simulink model "GuidanceLaw"  (R2023b)
settings: Solver=ode4  StartTime=0.0  StopTime=400  FixedStep=0.05  RelTol=1e-3
values from neighbouring files (symbols this model uses):
  APCMD_TYPE : value not decoded    [apDataDictionary.sldd]
  missionRoutePlan_struct = struct(      'validWpNum_u8', uint8(5),      'missionRoute_struct', repmat(wpDefault_struct, double(maxWpNum_u8), 1))    [initMissionRoutePlan_MC.m]
  MSSN_TYPE : value not decoded    [apDataDictionary.sldd]
  setPoint_struct = struct('lat_deg_d',double(31.200000),'lon_deg_d',double(121.500000),'alt_m_f',single(100),'yaw_deg_f',single(0))    [APTest.m]
undefined symbols (not defined in the file or in its folder): apParams
libraries: simulink x13, simulink_extras x3
(part 2 of 7)

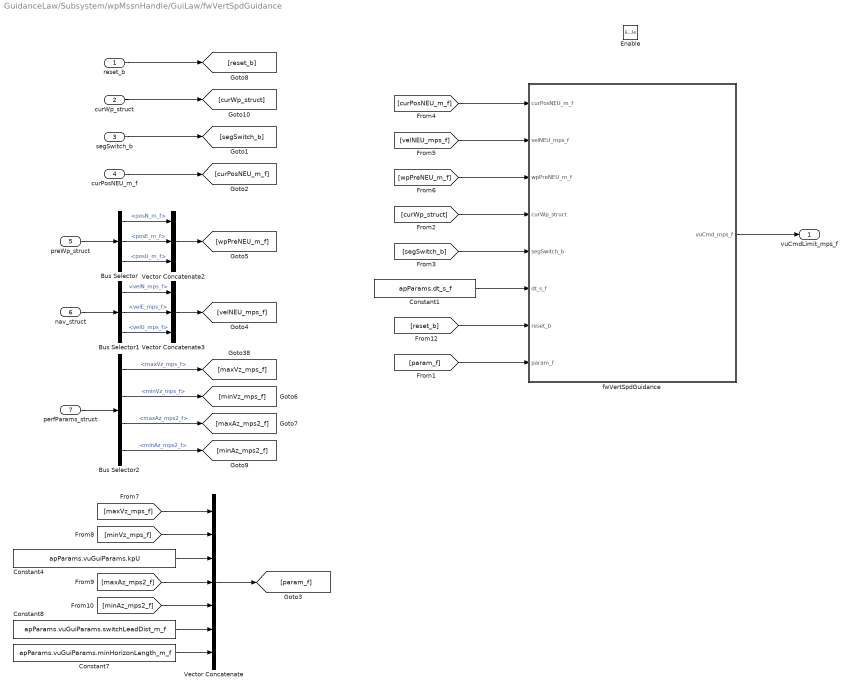
== system GuidanceLaw/Subsystem/wpMssnHandle/GuiLaw/fwVertSpdGuidance ==
  reset_b : Inport
  curWp_struct : Inport  Port=2
  segSwitch_b : Inport  Port=3
  curPosNEU_m_f : Inport  Port=4
  preWp_struct : Inport  Port=5
  nav_struct : Inport  Port=6
  perfParams_struct : Inport  Port=7
  Enable : EnablePort  StatesWhenEnabling=reset
  Bus Selector : BusSelector  OutputSignals=posN_m_f,posE_m_f,posU_m_f
  Bus Selector1 : BusSelector  OutputSignals=velN_mps_f,velE_mps_f,velU_mps_f
  Bus Selector2 : BusSelector  OutputSignals=maxVz_mps_f,minVz_mps_f,maxAz_mps2_f,minAz_mps2_f
  Constant1 : Constant  Value=apParams.dt_s_f  OutDataTypeStr=single
  Constant4 : Constant  Value=apParams.vuGuiParams.kpU  OutDataTypeStr=single
  Constant7 : Constant  Value=apParams.vuGuiParams.minHorizonLength_m_f  OutDataTypeStr=single
  Constant8 : Constant  Value=apParams.vuGuiParams.switchLeadDist_m_f  OutDataTypeStr=single
  Vector Concatenate : Concatenate  NumInputs=7
  Vector Concatenate2 : Concatenate  NumInputs=3
  Vector Concatenate3 : Concatenate  NumInputs=3
  fwVertSpdGuidance : MATLAB Function  TreatAsAtomicUnit=on
  vuCmdLimit_mps_f : Outport
  wires:
  fwVertSpdGuidance/1(vuCmd_mps_f) -> vuCmdLimit_mps_f/1
  Constant1/1 -> fwVertSpdGuidance/6(dt_s_f)
  reset_b/1 -> [reset_b]
  [reset_b] -> fwVertSpdGuidance/7(reset_b)
  Vector Concatenate/1 -> [param_f]
  [param_f] -> fwVertSpdGuidance/8(param_f)
  curWp_struct/1 -> [curWp_struct]
  [maxVz_mps_f] -> Vector Concatenate/1
  [minVz_mps_f] -> Vector Concatenate/2
  Constant4/1 -> Vector Concatenate/3
  [maxAz_mps2_f] -> Vector Concatenate/4
  [minAz_mps2_f] -> Vector Concatenate/5
  Constant7/1 -> Vector Concatenate/7
  Constant8/1 -> Vector Concatenate/6
  [curWp_struct] -> fwVertSpdGuidance/4(curWp_struct)
  segSwitch_b/1 -> [segSwitch_b]
  [segSwitch_b] -> fwVertSpdGuidance/5(segSwitch_b)
  curPosNEU_m_f/1 -> [curPosNEU_m_f]
  [curPosNEU_m_f] -> fwVertSpdGuidance/1(curPosNEU_m_f)
  [velNEU_mps_f] -> fwVertSpdGuidance/2(velNEU_mps_f)
  [wpPreNEU_m_f] -> fwVertSpdGuidance/3(wpPreNEU_m_f)
  preWp_struct/1 -> Bus Selector/1
  nav_struct/1 -> Bus Selector1/1
  Bus Selector/1 -> Vector Concatenate2/1  "<posN_m_f>"
  Bus Selector/2 -> Vector Concatenate2/2  "<posE_m_f>"
  Bus Selector/3 -> Vector Concatenate2/3  "<posU_m_f>"
  Vector Concatenate2/1 -> [wpPreNEU_m_f]
  Bus Selector1/1 -> Vector Concatenate3/1  "<velN_mps_f>"
  Bus Selector1/2 -> Vector Concatenate3/2  "<velE_mps_f>"
  Bus Selector1/3 -> Vector Concatenate3/3  "<velU_mps_f>"
  Vector Concatenate3/1 -> [velNEU_mps_f]
  perfParams_struct/1 -> Bus Selector2/1
  Bus Selector2/1 -> [maxVz_mps_f]  "<maxVz_mps_f>"
  Bus Selector2/2 -> [minVz_mps_f]  "<minVz_mps_f>"
  Bus Selector2/3 -> [maxAz_mps2_f]  "<maxAz_mps2_f>"
  Bus Selector2/4 -> [minAz_mps2_f]  "<minAz_mps2_f>"

== system GuidanceLaw/Subsystem/wpMssnHandle/GuiLaw/guiLawSelect ==
  flightPhase_enum : Inport
  preWp_struct : Inport  Port=2
  curWp_struct : Inport  Port=3
  guiLawSelect : MATLAB Function  TreatAsAtomicUnit=on
  guiLawType_u8 : Outport
  fwL1LineGui_b : Outport  Port=2
  fwL1CirGui_b : Outport  Port=3
  fwAirSpdGui_b : Outport  Port=4
  fwVertSpdGui_b : Outport  Port=5
  mcSpdGui_b : Outport  Port=6
  yawGui_b : Outport  Port=7
  segMssnType_u8 : Outport  Port=8
  tiltEnable_b : Outport  Port=9
  wires:
  guiLawSelect/1(guiLawType_u8) -> [guiLawType_u8]
  guiLawSelect/2(fwL1LineGui_b) -> [fwL1LineGui_b]
  guiLawSelect/3(fwL1CirGui_b) -> [fwL1CirGui_b]
  guiLawSelect/4(fwAirSpdGui_b) -> [fwAirSpdGui_b]
  guiLawSelect/5(fwVertSpdGui_b) -> [fwVertSpdGui_b]
  guiLawSelect/6(mcSpdGui_b) -> [mcSpdGui_b]
  guiLawSelect/7(yawGui_b) -> [yawGui_b]
  [flightPhase_enum] -> guiLawSelect/1(flightPhase_enum)
  [preWp_struct] -> guiLawSelect/2(preWp_struct)
  [curWp_struct] -> guiLawSelect/3(curWp_struct)
  flightPhase_enum/1 -> [flightPhase_enum]
  preWp_struct/1 -> [preWp_struct]
  curWp_struct/1 -> [curWp_struct]
  [guiLawType_u8] -> guiLawType_u8/1
  [fwL1LineGui_b] -> fwL1LineGui_b/1
  [fwL1CirGui_b] -> fwL1CirGui_b/1
  [fwAirSpdGui_b] -> fwAirSpdGui_b/1
  [fwVertSpdGui_b] -> fwVertSpdGui_b/1
  [mcSpdGui_b] -> mcSpdGui_b/1
  [yawGui_b] -> yawGui_b/1
  guiLawSelect/8(segMssnType_u8) -> [segMssnType_u8]
  [segMssnType_u8] -> segMssnType_u8/1
  guiLawSelect/9(tiltEnable_b) -> [tiltEnable_b]
  [tiltEnable_b] -> tiltEnable_b/1

== system GuidanceLaw/Subsystem/wpMssnHandle/GuiLaw/invaildGuidance ==
  nav_struct : Inport
  Bus Selector : BusSelector  OutputSignals=velN_mps_f,velE_mps_f,velU_mps_f,roll_deg_f,pitch_deg_f,yaw_deg_f
  NE2Body : Subsystem
  vuCmd_mps_f : Outport
  rollCmd_deg_f : Outport  Port=2
  pitchCmd_deg_f : Outport  Port=3
  yawCmd_deg_f : Outport  Port=4
  vyCmd_mps_f : Outport  Port=5
  vxCmd_mps_f : Outport  Port=6
  wires:
  nav_struct/1 -> Bus Selector/1
  Bus Selector/3 -> vuCmd_mps_f/1  "<velU_mps_f>"
  Bus Selector/4 -> rollCmd_deg_f/1  "<roll_deg_f>"
  Bus Selector/5 -> pitchCmd_deg_f/1  "<pitch_deg_f>"
  Bus Selector/6 -> [curYaw_deg_f], yawCmd_deg_f/1  "<yaw_deg_f>"
  Bus Selector/1 -> [curVn_mps_f]  "<velN_mps_f>"
  Bus Selector/2 -> [curVe_mps_f]  "<velE_mps_f>"
  NE2Body/1(vxCmd_mps_f) -> vxCmd_mps_f/1  "vxCmd_mps_f"
  NE2Body/2(vyCmd_mps_f) -> vyCmd_mps_f/1  "vyCmd_mps_f"
  [curYaw_deg_f] -> NE2Body/1(curYaw_deg_f)
  [curVe_mps_f] -> NE2Body/3(curVe_mps_f)
  [curVn_mps_f] -> NE2Body/2(curVn_mps_f)

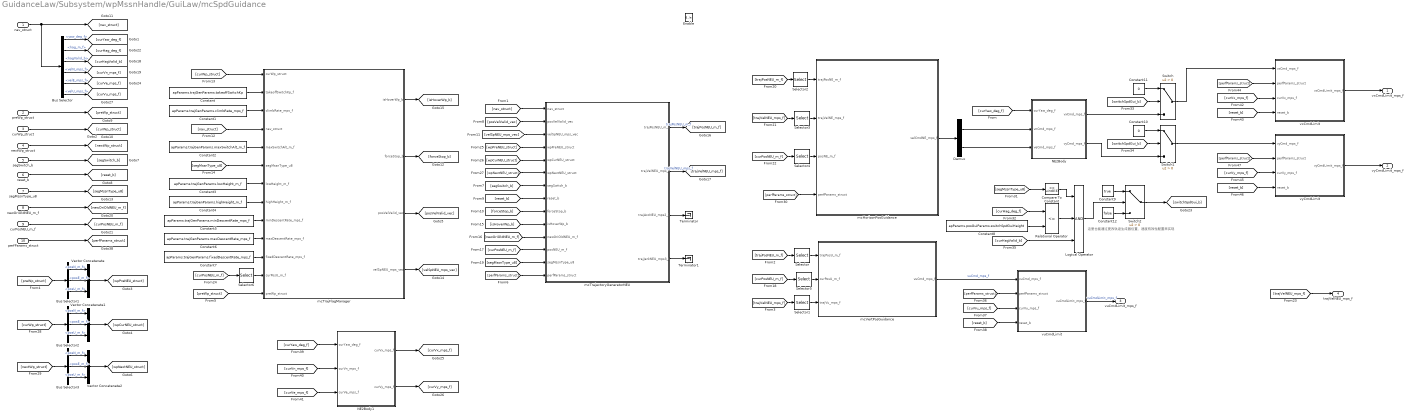
== system GuidanceLaw/Subsystem/wpMssnHandle/GuiLaw/mcSpdGuidance ==
  note: 这里也能通过更改轨迹生成器位置、速度有效性配置来实现
  nav_struct : Inport
  preWp_struct : Inport  Port=2
  curWp_struct : Inport  Port=3
  nextWp_struct : Inport  Port=4
  segSwitch_b : Inport  Port=5
  reset_b : Inport  Port=6
  segMssnType_u8 : Inport  Port=7
  newOriOldNEU_m_f : Inport  Port=8
  curPosNEU_m_f : Inport  Port=9
  perfParams_struct : Inport  Port=10
  Enable : EnablePort  StatesWhenEnabling=reset
  Bus Selector : BusSelector  OutputSignals=yaw_deg_f,hag_m_f,hagValid_b,velN_mps_f,velE_mps_f,velU_mps_f
  Bus Selector1 : BusSelector  OutputSignals=posN_m_f,posE_m_f,posU_m_f
  Bus Selector2 : BusSelector  OutputSignals=posN_m_f,posE_m_f,posU_m_f
  Bus Selector3 : BusSelector  OutputSignals=posN_m_f,posE_m_f,posU_m_f
  Compare To Constant : simulink/Logic and Bit Operations/Compare To Constant  relop===  const=uint8(3)  OutDataTypeStr=boolean
  Constant : Constant  Value=apParams.trajGenParams.takeoffSwitchKp  OutDataTypeStr=single
  Constant1 : Constant  Value=apParams.trajGenParams.climbRate_mps_f  OutDataTypeStr=single
  Constant10 : Constant  Value=0  OutDataTypeStr=single
  Constant11 : Constant  Value=0  OutDataTypeStr=single
  Constant12 : Constant  Value=false  OutDataTypeStr=boolean
  Constant2 : Constant  Value=apParams.trajGenParams.maxSwitchAlt_m_f  OutDataTypeStr=single
  Constant3 : Constant  Value=apParams.trajGenParams.lowHeight_m_f  OutDataTypeStr=single
  Constant4 : Constant  Value=apParams.trajGenParams.highHeight_m_f  OutDataTypeStr=single
  Constant5 : Constant  Value=apParams.trajGenParams.minDescentRate_mps_f  OutDataTypeStr=single
  Constant6 : Constant  Value=apParams.trajGenParams.maxDescentRate_mps_f  OutDataTypeStr=single
  Constant7 : Constant  Value=apParams.trajGenParams.fixedDescentRate_mps_f  OutDataTypeStr=single
  Constant8 : Constant  Value=apParams.posGuiParams.switchSpdGuiHeight  OutDataTypeStr=single
  Constant9 : Constant  Value=true  OutDataTypeStr=boolean
  Demux : Demux  Outputs=2
  Logical Operator : Logic  Inputs=3  AllPortsSameDT=off  OutDataTypeStr=boolean
  NE2Body : Subsystem
  NE2Body1 : Subsystem
  Relational Operator : RelationalOperator  Operator=<=  OutDataTypeStr=boolean  RndMeth=Simplest  InputSameDT=off
  Selector{,1,5..6} (4 alike) : Selector  InputPortWidth=3  IndexOptions=Index vector (dialog)  Indices=3  OutputSizes=1
  Selector2 : Selector  InputPortWidth=3  IndexOptions=Index vector (dialog)  Indices=[1 2]  OutputSizes=1
  Selector3 : Selector  InputPortWidth=3  IndexOptions=Index vector (dialog)  Indices=[1 2]  OutputSizes=1
  Selector4 : Selector  InputPortWidth=3  IndexOptions=Index vector (dialog)  Indices=[1 2]  OutputSizes=1
  Switch : Switch  Criteria=u2 > Threshold  SaturateOnIntegerOverflow=off  InputSameDT=off
  Switch1 : Switch  Criteria=u2 > Threshold  SaturateOnIntegerOverflow=off  InputSameDT=off
  Switch2 : Switch  Criteria=u2 > Threshold  SaturateOnIntegerOverflow=off  InputSameDT=off
  Terminator : Terminator
  Terminator1 : Terminator
  Vector Concatenate : Concatenate  NumInputs=3
  Vector Concatenate1 : Concatenate  NumInputs=3
  Vector Concatenate2 : Concatenate  NumInputs=3
  mcHorizonPosGuidance : Subsystem
  mcTrajFlagManager : MATLAB Function  TreatAsAtomicUnit=on
  mcTrajectoryGeneratorNEU : Subsystem
  mcVertPosGuidance : Subsystem
  vuCmdLimit : Subsystem
  vxCmdLimit : Subsystem
  vyCmdLimit : Subsystem
  vxCmdLimit_mps_f : Outport
  vyCmdLimit_mps_f : Outport  Port=2
  vuCmdLimit_mps_f : Outport  Port=3
  trajVelNEU_mps_f : Outport  Port=4
  wires:
  mcVertPosGuidance/1(vuCmd_mps_f) -> vuCmdLimit/1(vuCmd_mps_f)  "vuCmd_mps_f"
  NE2Body/1(vxCmd_mps_f) -> Switch/3
  mcHorizonPosGuidance/1(velCmdNE_mps_f) -> Demux/1
  Demux/1 -> NE2Body/2(vnCmd_mps_f)
  Demux/2 -> NE2Body/3(veCmd_mps_f)
  nav_struct/1 -> Bus Selector/1, [nav_struct]
  Bus Selector/1 -> [curYaw_deg_f]  "<yaw_deg_f>"
  [curYaw_deg_f] -> NE2Body/1(curYaw_deg_f)
  curWp_struct/1 -> [curWp_struct]
  preWp_struct/1 -> [preWp_struct]
  nextWp_struct/1 -> [nextWp_struct]
  [nav_struct] -> mcTrajectoryGeneratorNEU/1(nav_struct)
  segSwitch_b/1 -> [segSwitch_b]
  [segSwitch_b] -> mcTrajectoryGeneratorNEU/7(segSwitch_b)
  reset_b/1 -> [reset_b]
  [reset_b] -> mcTrajectoryGeneratorNEU/8(reset_b)
  [posVelValid_vec] -> mcTrajectoryGeneratorNEU/2(posVelValid_vec)
  mcTrajFlagManager/3(posVelValid_vec) -> [posVelValid_vec]
  [forceStop_b] -> mcTrajectoryGeneratorNEU/9(forceStop_b)
  [velSpNEU_mps_vec] -> mcTrajectoryGeneratorNEU/3(velSpNEU_mps_vec)
  [nav_struct] -> mcTrajFlagManager/4(nav_struct)
  [curWp_struct] -> mcTrajFlagManager/1(curWp_struct)
  Constant/1 -> mcTrajFlagManager/2(takeoffSwitchKp_f)
  Constant1/1 -> mcTrajFlagManager/3(climbRate_mps_f)
  Constant2/1 -> mcTrajFlagManager/5(maxSwitchAlt_m_f)
  mcTrajFlagManager/2(forceStop_b) -> [forceStop_b]
  segMssnType_u8/1 -> [segMssnType_u8]
  [segMssnType_u8] -> mcTrajFlagManager/6(segMssnType_u8)
  mcTrajFlagManager/4(velSpNEU_mps_vec) -> [velSpNEU_mps_vec]
  Constant3/1 -> mcTrajFlagManager/7(lowHeight_m_f)
  Constant4/1 -> mcTrajFlagManager/8(highHeight_m_f)
  Constant5/1 -> mcTrajFlagManager/9(minDescentRate_mps_f)
  Constant6/1 -> mcTrajFlagManager/10(maxDescentRate_mps_f)
  Constant7/1 -> mcTrajFlagManager/11(fixedDescentRate_mps_f)
  mcTrajFlagManager/1(isHoverWp_b) -> [isHoverWp_b]
  [isHoverWp_b] -> mcTrajectoryGeneratorNEU/10(isHoverWp_b)
  [newOriOldNEU_m_f] -> mcTrajectoryGeneratorNEU/11(newOriOldNEU_m_f)
  [curPosNEU_m_f] -> mcTrajectoryGeneratorNEU/12(posNEU_m_f)
  mcTrajectoryGeneratorNEU/1(trajPosNEU_m_f) -> [trajPosNEU_m_f]  "trajPosNEU_m_f"
  mcTrajectoryGeneratorNEU/2(trajVelNEU_mps_f) -> [trajVelNEU_mps_f]  "trajVelNEU_mps_f"
  mcTrajectoryGeneratorNEU/3(trajAccNEU_mps2_f) -> Terminator/1
  mcTrajectoryGeneratorNEU/4(trajJerkNEU_mps3_f) -> Terminator1/1
  newOriOldNEU_m_f/1 -> [newOriOldNEU_m_f]
  curPosNEU_m_f/1 -> [curPosNEU_m_f]
  [trajPosNEU_m_f] -> Selector/1
  Selector/1 -> mcVertPosGuidance/1(trajPosU_m_f)
  [trajVelNEU_mps_f] -> Selector1/1
  Selector1/1 -> mcVertPosGuidance/3(trajVu_mps_f)
  [curPosNEU_m_f] -> Selector5/1
  [segMssnType_u8] -> mcTrajectoryGeneratorNEU/13(segMssnType_u8)
  [trajPosNEU_m_f] -> Selector2/1
  Selector2/1 -> mcHorizonPosGuidance/1(trajPosNE_m_f)
  [trajVelNEU_mps_f] -> Selector3/1
  Selector3/1 -> mcHorizonPosGuidance/2(trajVelNE_mps_f)
  [curPosNEU_m_f] -> Selector4/1
  Selector4/1 -> mcHorizonPosGuidance/3(posNE_m_f)
  [trajVelNEU_mps_f] -> trajVelNEU_mps_f/1
  Selector5/1 -> mcVertPosGuidance/2(curPosU_m_f)
  [curPosNEU_m_f] -> Selector6/1
  Selector6/1 -> mcTrajFlagManager/12(curPosU_m_f)
  [preWp_struct] -> Bus Selector1/1
  Bus Selector1/1 -> Vector Concatenate/1  "<posN_m_f>"
  Bus Selector1/2 -> Vector Concatenate/2  "<posE_m_f>"
  Bus Selector1/3 -> Vector Concatenate/3  "<posU_m_f>"
  Vector Concatenate/1 -> [wpPreNEU_struct]
  [wpPreNEU_struct] -> mcTrajectoryGeneratorNEU/4(wpPreNEU_struct)
  [wpCurNEU_struct] -> mcTrajectoryGeneratorNEU/5(wpCurNEU_struct)
  [wpNextNEU_struct] -> mcTrajectoryGeneratorNEU/6(wpNextNEU_struct)
  Bus Selector2/3 -> Vector Concatenate1/3  "<posU_m_f>"
  Bus Selector2/2 -> Vector Concatenate1/2  "<posE_m_f>"
  Bus Selector2/1 -> Vector Concatenate1/1  "<posN_m_f>"
  Vector Concatenate1/1 -> [wpCurNEU_struct]
  [curWp_struct] -> Bus Selector2/1
  Bus Selector3/2 -> Vector Concatenate2/2  "<posE_m_f>"
  [nextWp_struct] -> Bus Selector3/1
  Bus Selector3/1 -> Vector Concatenate2/1  "<posN_m_f>"
  Bus Selector3/3 -> Vector Concatenate2/3  "<posU_m_f>"
  Vector Concatenate2/1 -> [wpNextNEU_struct]
  [preWp_struct] -> mcTrajFlagManager/13(preWp_struct)
  perfParams_struct/1 -> [perfParams_struct]
  [perfParams_struct] -> mcTrajectoryGeneratorNEU/14(perfParams_struct)
  [perfParams_struct] -> mcHorizonPosGuidance/4(perfParams_struct)
  Switch/1 -> vxCmdLimit/1(vxCmd_mps_f)
  NE2Body/2(vyCmd_mps_f) -> Switch1/3
  Constant10/1 -> Switch1/1
  Constant11/1 -> Switch/1
  [segMssnType_u8] -> Compare To Constant/1
  Compare To Constant/1 -> Logical Operator/1
  [curHag_deg_f] -> Relational Operator/1
  Bus Selector/2 -> [curHag_deg_f]  "<hag_m_f>"
  Constant8/1 -> Relational Operator/2
  Relational Operator/1 -> Logical Operator/2
  Logical Operator/1 -> Switch2/2
  Constant9/1 -> Switch2/1
  Constant12/1 -> Switch2/3
  Switch2/1 -> [switchSpdGui_b]
  [switchSpdGui_b] -> Switch/2
  [switchSpdGui_b] -> Switch1/2
  Bus Selector/3 -> [curHagValid_b]  "<hagValid_b>"
  [curHagValid_b] -> Logical Operator/3
  vuCmdLimit/1(vuCmdLimit_mps_f) -> vuCmdLimit_mps_f/1  "vuCmdLimit_mps_f"
  [perfParams_struct] -> vuCmdLimit/2(perfParams_struct)
  [curVu_mps_f] -> vuCmdLimit/3(curVu_mps_f)
  [reset_b] -> vuCmdLimit/4(reset_b)
  vxCmdLimit/1(vxCmdLimit_mps_f) -> vxCmdLimit_mps_f/1
  [curYaw_deg_f] -> NE2Body1/1(curYaw_deg_f)
  Bus Selector/4 -> [curVn_mps_f]  "<velN_mps_f>"
  Bus Selector/5 -> [curVe_mps_f]  "<velE_mps_f>"
  [curVn_mps_f] -> NE2Body1/2(curVn_mps_f)
  [curVe_mps_f] -> NE2Body1/3(curVe_mps_f)
  NE2Body1/1(curVx_mps_f) -> [curVx_mps_f]
  NE2Body1/2(curVy_mps_f) -> [curVy_mps_f]
  [curVx_mps_f] -> vxCmdLimit/3(curVx_mps_f)
  [reset_b] -> vxCmdLimit/4(reset_b)
  [perfParams_struct] -> vxCmdLimit/2(perfParams_struct)
  [reset_b] -> vyCmdLimit/4(reset_b)
  [curVy_mps_f] -> vyCmdLimit/3(curVy_mps_f)
  [perfParams_struct] -> vyCmdLimit/2(perfParams_struct)
  Switch1/1 -> vyCmdLimit/1(vyCmd_mps_f)
  vyCmdLimit/1(vyCmdLimit_mps_f) -> vyCmdLimit_mps_f/1
  Bus Selector/6 -> [curVu_mps_f]  "<velU_mps_f>"

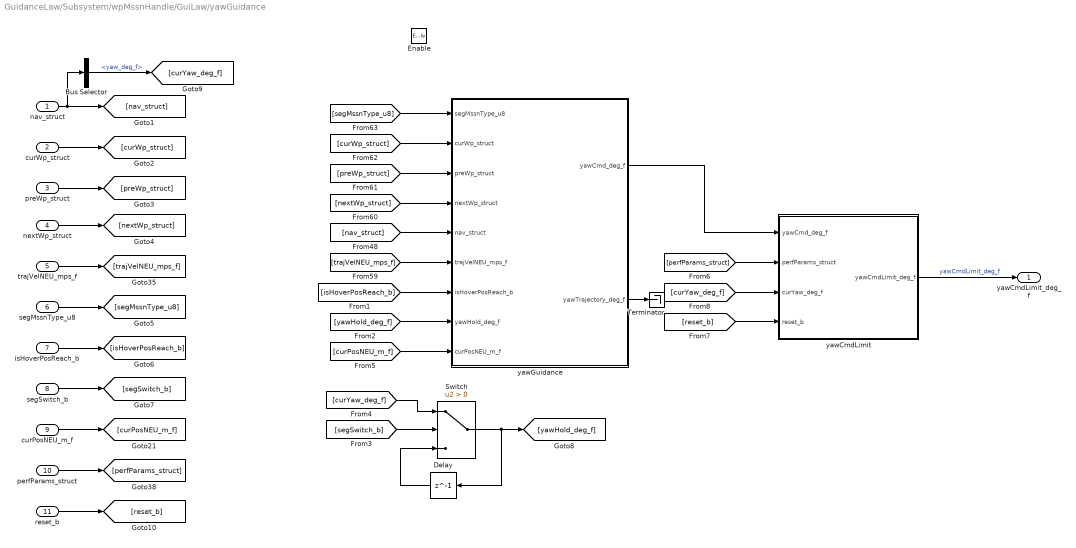
== system GuidanceLaw/Subsystem/wpMssnHandle/GuiLaw/yawGuidance ==
  nav_struct : Inport
  curWp_struct : Inport  Port=2
  preWp_struct : Inport  Port=3
  nextWp_struct : Inport  Port=4
  trajVelNEU_mps_f : Inport  Port=5
  segMssnType_u8 : Inport  Port=6
  isHoverPosReach_b : Inport  Port=7
  segSwitch_b : Inport  Port=8
  curPosNEU_m_f : Inport  Port=9
  perfParams_struct : Inport  Port=10
  reset_b : Inport  Port=11
  Enable : EnablePort  StatesWhenEnabling=reset
  Bus Selector : BusSelector  OutputSignals=yaw_deg_f
  Delay : Delay  DelayLength=1
  Switch : Switch  Criteria=u2 > Threshold  SaturateOnIntegerOverflow=off  InputSameDT=off
  Terminator : Terminator
  yawCmdLimit : Subsystem
  yawGuidance : MATLAB Function  TreatAsAtomicUnit=on
  yawCmdLimit_deg_f : Outport
  wires:
  trajVelNEU_mps_f/1 -> [trajVelNEU_mps_f]
  nav_struct/1 -> Bus Selector/1, [nav_struct]
  curWp_struct/1 -> [curWp_struct]
  preWp_struct/1 -> [preWp_struct]
  nextWp_struct/1 -> [nextWp_struct]
  segMssnType_u8/1 -> [segMssnType_u8]
  [nav_struct] -> yawGuidance/5(nav_struct)
  [nextWp_struct] -> yawGuidance/4(nextWp_struct)
  [preWp_struct] -> yawGuidance/3(preWp_struct)
  [curWp_struct] -> yawGuidance/2(curWp_struct)
  [segMssnType_u8] -> yawGuidance/1(segMssnType_u8)
  [trajVelNEU_mps_f] -> yawGuidance/6(trajVelNEU_mps_f)
  isHoverPosReach_b/1 -> [isHoverPosReach_b]
  [isHoverPosReach_b] -> yawGuidance/7(isHoverPosReach_b)
  segSwitch_b/1 -> [segSwitch_b]
  [yawHold_deg_f] -> yawGuidance/8(yawHold_deg_f)
  [segSwitch_b] -> Switch/2
  Switch/1 -> Delay/1, [yawHold_deg_f]
  Bus Selector/1 -> [curYaw_deg_f]  "<yaw_deg_f>"
  [curYaw_deg_f] -> Switch/1
  Delay/1 -> Switch/3
  curPosNEU_m_f/1 -> [curPosNEU_m_f]
  [curPosNEU_m_f] -> yawGuidance/9(curPosNEU_m_f)
  yawCmdLimit/1(yawCmdLimit_deg_f) -> yawCmdLimit_deg_f/1  "yawCmdLimit_deg_f"
  yawGuidance/1(yawCmd_deg_f) -> yawCmdLimit/1(yawCmd_deg_f)
  perfParams_struct/1 -> [perfParams_struct]
  [perfParams_struct] -> yawCmdLimit/2(perfParams_struct)
  reset_b/1 -> [reset_b]
  [reset_b] -> yawCmdLimit/4(reset_b)
  [curYaw_deg_f] -> yawCmdLimit/3(curYaw_deg_f)
  yawGuidance/2(yawTrajectory_deg_f) -> Terminator/1

== system GuidanceLaw/Subsystem/wpMssnHandle/WaypointArrivalState/cirJudge ==
  curPosNEU_m_f : Inport
  curWp_struct : Inport  Port=2
  nextWp_struct : Inport  Port=3
  reset_b : Inport  Port=4
  Enable : EnablePort  StatesWhenEnabling=reset
  Bus Selector1 : BusSelector  OutputSignals=posN_m_f,posE_m_f,posU_m_f,timeOrCount_u16,arrivalCond_u8
  Bus Selector2 : BusSelector  OutputSignals=posN_m_f,posE_m_f,posU_m_f
  Constant1 : Constant  Value=apParams.cirJudge.cirAltTolerance_m_f  OutDataTypeStr=single
  Constant21 : Constant  Value=apParams.dt_s_f  OutDataTypeStr=single
  Constant5 : Constant  Value=apParams.cirJudge.cirExitTolerance_deg_f  OutDataTypeStr=single
  MATLAB Function : MATLAB Function  TreatAsAtomicUnit=on
  MATLAB Function1 : MATLAB Function  Commented=on  TreatAsAtomicUnit=on
  Vector Concatenate1 : Concatenate  NumInputs=3
  Vector Concatenate2 : Concatenate  NumInputs=3
  cirJudge_b : Outport
  wires:
  MATLAB Function/1(cirJudge_b) -> cirJudge_b/1
  curPosNEU_m_f/1 -> MATLAB Function/1(curPosNEU_m_f)
  nextWp_struct/1 -> Bus Selector2/1
  Bus Selector1/1 -> Vector Concatenate1/1  "<posN_m_f>"
  Bus Selector1/2 -> Vector Concatenate1/2  "<posE_m_f>"
  Vector Concatenate1/1 -> [curWpNEU_m_f]
  Bus Selector2/2 -> Vector Concatenate2/2  "<posE_m_f>"
  Vector Concatenate2/1 -> [nextWpNEU_m_f]
  Bus Selector2/1 -> Vector Concatenate2/1  "<posN_m_f>"
  curWp_struct/1 -> Bus Selector1/1
  [curWpNEU_m_f] -> MATLAB Function/2(curWpNEU_m_f)
  [nextWpNEU_m_f] -> MATLAB Function/3(nextWpNEU_m_f)
  reset_b/1 -> MATLAB Function/9(reset_b)
  Constant5/1 -> MATLAB Function/6(cirExitTolerance_deg_f)
  Constant21/1 -> MATLAB Function/8(dt_s_f)
  Constant1/1 -> MATLAB Function/7(cirAltTolerance_m_f)
  Bus Selector1/4 -> [timeOrCount_u16]  "<timeOrCount_u16>"
  Bus Selector1/5 -> [arrivalCond_u8]  "<arrivalCond_u8>"
  [arrivalCond_u8] -> MATLAB Function/4(arrivalCond_u8)
  [timeOrCount_u16] -> MATLAB Function/5(timeOrCount_u16)
  Bus Selector1/3 -> Vector Concatenate1/3  "<posU_m_f>"
  Bus Selector2/3 -> Vector Concatenate2/3  "<posU_m_f>"

== system GuidanceLaw/Subsystem/wpMssnHandle/WaypointArrivalState/fwLineJudge ==
  curPosNEU_m_f : Inport
  reset_b : Inport  Port=2
  preWp_struct : Inport  Port=3
  curWp_struct : Inport  Port=4
  nextWp_struct : Inport  Port=5
  Enable : EnablePort  StatesWhenEnabling=reset
  Constant1 : Constant  Value=apParams.fwLineJudge.minJudgeDist_m_f  OutDataTypeStr=single
  Constant2 : Constant  Value=apParams.fwLineJudge.maxJudgeDist_m_f  OutDataTypeStr=single
  Constant3 : Constant  Value=apParams.fwLineJudge.segmentLimitRatio_f  OutDataTypeStr=single
  Constant4 : Constant  Value=apParams.G_mps2_f  OutDataTypeStr=single
  Constant5 : Constant  Value=apParams.fwLineJudge.effectRollRate_dps_f  OutDataTypeStr=single
  Constant6 : Constant  Value=apParams.airSpdGuiParams.cruiseAirSpd_mps_f  OutDataTypeStr=single
  Constant7 : Constant  Value=apParams.fwLineJudge.turnRollPlan_deg_f  OutDataTypeStr=single
  Constant8 : Constant  Value=apParams.fwLineJudge.judgeDistMargin_f  OutDataTypeStr=single
  JudgeAlgorithm : MATLAB Function  TreatAsAtomicUnit=on
  Selector : Selector  InputPortWidth=3  IndexOptions=Index vector (dialog)  Indices=[1 2]  OutputSizes=1
  fwLineJudge_b : Outport
  wires:
  JudgeAlgorithm/1(fwLineJudge_b) -> fwLineJudge_b/1
  reset_b/1 -> JudgeAlgorithm/11(reset_b)
  Constant3/1 -> JudgeAlgorithm/10(segmentLimitRatio_f)
  Constant2/1 -> JudgeAlgorithm/9(maxJudgeDist_m_f)
  Constant1/1 -> JudgeAlgorithm/8(minJudgeDist_m_f)
  Constant5/1 -> JudgeAlgorithm/6(effectRollRate_dps_f)
  Constant4/1 -> JudgeAlgorithm/12(G_mps2_f)
  Selector/1 -> JudgeAlgorithm/1(curPosNE_m_f)
  curPosNEU_m_f/1 -> Selector/1
  preWp_struct/1 -> [preWp_struct]
  curWp_struct/1 -> [curWp_struct]
  nextWp_struct/1 -> [nextWp_struct]
  [preWp_struct] -> JudgeAlgorithm/2(preWp_struct)
  [curWp_struct] -> JudgeAlgorithm/3(curWp_struct)
  [nextWp_struct] -> JudgeAlgorithm/4(nextWp_struct)
  Constant7/1 -> JudgeAlgorithm/5(turnRollPlan_deg_f)
  Constant6/1 -> JudgeAlgorithm/13(cruiseAirSpd_mps_f)
  Constant8/1 -> JudgeAlgorithm/7(judgeDistMargin_f)

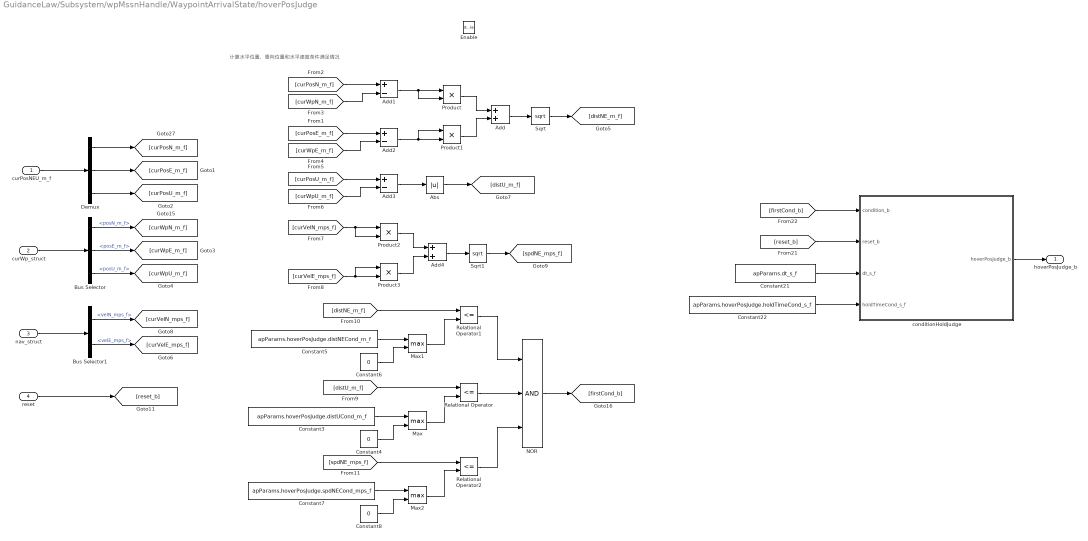
== system GuidanceLaw/Subsystem/wpMssnHandle/WaypointArrivalState/hoverPosJudge ==
  note: 计算水平位置、垂向位置和水平速度条件满足情况
  curPosNEU_m_f : Inport
  curWp_struct : Inport  Port=2
  nav_struct : Inport  Port=3
  reset : Inport  Port=4
  Enable : EnablePort  StatesWhenEnabling=reset
  Abs : Abs  SaturateOnIntegerOverflow=off
  Add : Sum
  Add1 : Sum  Inputs=+-
  Add2 : Sum  Inputs=+-
  Add3 : Sum  Inputs=+-
  Add4 : Sum
  Bus Selector : BusSelector  OutputSignals=posN_m_f,posE_m_f,posU_m_f
  Bus Selector1 : BusSelector  OutputSignals=velN_mps_f,velE_mps_f
  Constant21 : Constant  Value=apParams.dt_s_f  OutDataTypeStr=single
  Constant22 : Constant  Value=apParams.hoverPosJudge.holdTimeCond_s_f  OutDataTypeStr=single
  Constant3 : Constant  Value=apParams.hoverPosJudge.distUCond_m_f  OutDataTypeStr=single
  Constant4 : Constant  Value=0  OutDataTypeStr=single
  Constant5 : Constant  Value=apParams.hoverPosJudge.distNECond_m_f  OutDataTypeStr=single
  Constant6 : Constant  Value=0  OutDataTypeStr=single
  Constant7 : Constant  Value=apParams.hoverPosJudge.spdNECond_mps_f  OutDataTypeStr=single
  Constant8 : Constant  Value=0  OutDataTypeStr=single
  Demux : Demux  Outputs=3
  Max : MinMax  Function=max  Inputs=2
  Max1 : MinMax  Function=max  Inputs=2
  Max2 : MinMax  Function=max  Inputs=2
  NOR : Logic  Inputs=3  IconShape=distinctive  AllPortsSameDT=off  OutDataTypeStr=boolean
  Product{,1..3} (4 alike) : Product
  Relational Operator : RelationalOperator  Operator=<=  OutDataTypeStr=boolean  RndMeth=Simplest  InputSameDT=off
  Relational Operator1 : RelationalOperator  Operator=<=  OutDataTypeStr=boolean  RndMeth=Simplest  InputSameDT=off
  Relational Operator2 : RelationalOperator  Operator=<=  OutDataTypeStr=boolean  RndMeth=Simplest  InputSameDT=off
  Sqrt : Sqrt
  Sqrt1 : Sqrt
  conditionHoldJudge : MATLAB Function  TreatAsAtomicUnit=on
  hoverPosJudge_b : Outport
  wires:
  curPosNEU_m_f/1 -> Demux/1
  Demux/1 -> [curPosN_m_f]
  Demux/2 -> [curPosE_m_f]
  Demux/3 -> [curPosU_m_f]
  curWp_struct/1 -> Bus Selector/1
  Bus Selector/1 -> [curWpN_m_f]  "<posN_m_f>"
  Bus Selector/2 -> [curWpE_m_f]  "<posE_m_f>"
  Bus Selector/3 -> [curWpU_m_f]  "<posU_m_f>"
  Add1/1 -> Product/2, Product/1
  Add2/1 -> Product1/1, Product1/2
  Product/1 -> Add/1
  Product1/1 -> Add/2
  Add/1 -> Sqrt/1
  Sqrt/1 -> [distNE_m_f]
  [curPosN_m_f] -> Add1/1
  [curWpN_m_f] -> Add1/2
  nav_struct/1 -> Bus Selector1/1
  Bus Selector1/1 -> [curVelN_mps_f]  "<velN_mps_f>"
  Bus Selector1/2 -> [curVelE_mps_f]  "<velE_mps_f>"
  [curPosE_m_f] -> Add2/1
  [curWpE_m_f] -> Add2/2
  [curPosU_m_f] -> Add3/1
  [curWpU_m_f] -> Add3/2
  Add3/1 -> Abs/1
  Abs/1 -> [distU_m_f]
  Add4/1 -> Sqrt1/1
  [curVelN_mps_f] -> Product2/2, Product2/1
  Product2/1 -> Add4/1
  [curVelE_mps_f] -> Product3/1, Product3/2
  Product3/1 -> Add4/2
  Sqrt1/1 -> [spdNE_mps_f]
  Constant3/1 -> Max/1
  Constant4/1 -> Max/2
  [distU_m_f] -> Relational Operator/1
  Max/1 -> Relational Operator/2
  Relational Operator/1 -> NOR/2
  [distNE_m_f] -> Relational Operator1/1
  Max1/1 -> Relational Operator1/2
  Relational Operator1/1 -> NOR/1
  Constant6/1 -> Max1/2
  Constant5/1 -> Max1/1
  Constant8/1 -> Max2/2
  [spdNE_mps_f] -> Relational Operator2/1
  Max2/1 -> Relational Operator2/2
  Constant7/1 -> Max2/1
  Relational Operator2/1 -> NOR/3
  reset/1 -> [reset_b]
  NOR/1 -> [firstCond_b]
  conditionHoldJudge/1(hoverPosJudge_b) -> hoverPosJudge_b/1
  Constant21/1 -> conditionHoldJudge/3(dt_s_f)
  Constant22/1 -> conditionHoldJudge/4(holdTimeCond_s_f)
  [reset_b] -> conditionHoldJudge/2(reset_b)
  [firstCond_b] -> conditionHoldJudge/1(condition_b)

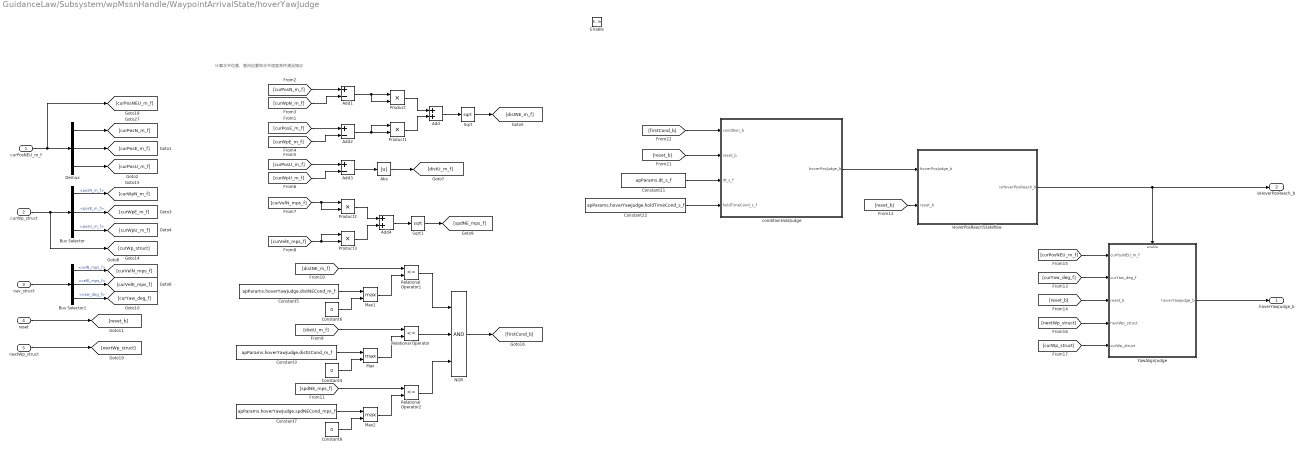
== system GuidanceLaw/Subsystem/wpMssnHandle/WaypointArrivalState/hoverYawJudge ==
  note: 计算水平位置、垂向位置和水平速度条件满足情况
  curPosNEU_m_f : Inport
  curWp_struct : Inport  Port=2
  nav_struct : Inport  Port=3
  reset : Inport  Port=4
  nextWp_struct : Inport  Port=5
  Enable : EnablePort  StatesWhenEnabling=reset
  Abs : Abs  SaturateOnIntegerOverflow=off
  Add : Sum
  Add1 : Sum  Inputs=+-
  Add2 : Sum  Inputs=+-
  Add3 : Sum  Inputs=+-
  Add4 : Sum
  Bus Selector : BusSelector  OutputSignals=posN_m_f,posE_m_f,posU_m_f
  Bus Selector1 : BusSelector  OutputSignals=velN_mps_f,velE_mps_f,yaw_deg_f
  Constant21 : Constant  Value=apParams.dt_s_f  OutDataTypeStr=single
  Constant22 : Constant  Value=apParams.hoverYawJudge.holdTimeCond_s_f  OutDataTypeStr=single
  Constant3 : Constant  Value=apParams.hoverYawJudge.distUCond_m_f  OutDataTypeStr=single
  Constant4 : Constant  Value=0  OutDataTypeStr=single
  Constant5 : Constant  Value=apParams.hoverYawJudge.distNECond_m_f  OutDataTypeStr=single
  Constant6 : Constant  Value=0  OutDataTypeStr=single
  Constant7 : Constant  Value=apParams.hoverYawJudge.spdNECond_mps_f  OutDataTypeStr=single
  Constant8 : Constant  Value=0  OutDataTypeStr=single
  Demux : Demux  Outputs=3
  HoverPosReachStateflow : Stateflow chart  TreatAsAtomicUnit=on
  Max : MinMax  Function=max  Inputs=2
  Max1 : MinMax  Function=max  Inputs=2
  Max2 : MinMax  Function=max  Inputs=2
  NOR : Logic  Inputs=3  IconShape=distinctive  AllPortsSameDT=off  OutDataTypeStr=boolean
  Product{,1..3} (4 alike) : Product
  Relational Operator : RelationalOperator  Operator=<=  OutDataTypeStr=boolean  RndMeth=Simplest  InputSameDT=off
  Relational Operator1 : RelationalOperator  Operator=<=  OutDataTypeStr=boolean  RndMeth=Simplest  InputSameDT=off
  Relational Operator2 : RelationalOperator  Operator=<=  OutDataTypeStr=boolean  RndMeth=Simplest  InputSameDT=off
  Sqrt : Sqrt
  Sqrt1 : Sqrt
  YawAlignJudge : Subsystem
  conditionHoldJudge : MATLAB Function  TreatAsAtomicUnit=on
  hoverYawJudge_b : Outport
  isHoverPosReach_b : Outport  Port=2
  wires:
  Product/1 -> Add/1
  [curPosN_m_f] -> Add1/1
  reset/1 -> [reset_b]
  Add3/1 -> Abs/1
  Add1/1 -> Product/2, Product/1
  Demux/3 -> [curPosU_m_f]
  nav_struct/1 -> Bus Selector1/1
  Bus Selector/3 -> [curWpU_m_f]  "<posU_m_f>"
  Demux/1 -> [curPosN_m_f]
  NOR/1 -> [firstCond_b]
  Product1/1 -> Add/2
  Demux/2 -> [curPosE_m_f]
  [curWpU_m_f] -> Add3/2
  [curWpN_m_f] -> Add1/2
  Sqrt/1 -> [distNE_m_f]
  Max1/1 -> Relational Operator1/2
  curPosNEU_m_f/1 -> [curPosNEU_m_f], Demux/1
  Constant4/1 -> Max/2
  [curWpE_m_f] -> Add2/2
  Max2/1 -> Relational Operator2/2
  Bus Selector/2 -> [curWpE_m_f]  "<posE_m_f>"
  Relational Operator1/1 -> NOR/1
  Relational Operator2/1 -> NOR/3
  Constant7/1 -> Max2/1
  Abs/1 -> [distU_m_f]
  Constant3/1 -> Max/1
  Bus Selector/1 -> [curWpN_m_f]  "<posN_m_f>"
  [curPosE_m_f] -> Add2/1
  Sqrt1/1 -> [spdNE_mps_f]
  [curPosU_m_f] -> Add3/1
  [spdNE_mps_f] -> Relational Operator2/1
  Add2/1 -> Product1/1, Product1/2
  Constant8/1 -> Max2/2
  Constant6/1 -> Max1/2
  [distNE_m_f] -> Relational Operator1/1
  [distU_m_f] -> Relational Operator/1
  curWp_struct/1 -> [curWp_struct], Bus Selector/1
  Max/1 -> Relational Operator/2
  Bus Selector1/1 -> [curVelN_mps_f]  "<velN_mps_f>"
  Relational Operator/1 -> NOR/2
  Product3/1 -> Add4/2
  [curVelE_mps_f] -> Product3/1, Product3/2
  Add/1 -> Sqrt/1
  Product2/1 -> Add4/1
  Bus Selector1/2 -> [curVelE_mps_f]  "<velE_mps_f>"
  [curVelN_mps_f] -> Product2/2, Product2/1
  Add4/1 -> Sqrt1/1
  Constant5/1 -> Max1/1
  [firstCond_b] -> conditionHoldJudge/1(condition_b)
  [reset_b] -> conditionHoldJudge/2(reset_b)
  conditionHoldJudge/1(hoverPosJudge_b) -> HoverPosReachStateflow/1(hoverPosJudge_b)
  Constant22/1 -> conditionHoldJudge/4(holdTimeCond_s_f)
  Constant21/1 -> conditionHoldJudge/3(dt_s_f)
  [reset_b] -> HoverPosReachStateflow/2(reset_b)
  HoverPosReachStateflow/1(isHoverPosReach_b) -> isHoverPosReach_b/1, YawAlignJudge/Enable
  YawAlignJudge/1(hoverYawJudge_b) -> hoverYawJudge_b/1
  Bus Selector1/3 -> [curYaw_deg_f]  "<yaw_deg_f>"
  nextWp_struct/1 -> [nextWp_struct]
  [curPosNEU_m_f] -> YawAlignJudge/1(curPosNEU_m_f)
  [curYaw_deg_f] -> YawAlignJudge/2(curYaw_deg_f)
  [reset_b] -> YawAlignJudge/3(reset_b)
  [nextWp_struct] -> YawAlignJudge/4(nextWp_struct)
  [curWp_struct] -> YawAlignJudge/5(curWp_struct)

== system GuidanceLaw/Subsystem/wpMssnHandle/WaypointArrivalState/mcLineJudge ==
  curPosNEU_m_f : Inport
  reset_b : Inport  Port=2
  preWp_struct : Inport  Port=3
  curWp_struct : Inport  Port=4
  nextWp_struct : Inport  Port=5
  perfParams_struct : Inport  Port=6
  Enable : EnablePort  StatesWhenEnabling=reset
  Abs : Abs  SaturateOnIntegerOverflow=off
  Bus Selector : BusSelector  OutputSignals=posN_m_f,posE_m_f
  Bus Selector1 : BusSelector  OutputSignals=posN_m_f,posE_m_f
  Bus Selector2 : BusSelector  OutputSignals=posN_m_f,posE_m_f
  Bus Selector3 : BusSelector  OutputSignals=maxAy_mps2_f
  Constant1 : Constant  Value=apParams.mcLineJudge.minJudgeDist_m_f  OutDataTypeStr=single
  Constant2 : Constant  Value=apParams.mcLineJudge.maxJudgeDist_m_f  OutDataTypeStr=single
  Constant3 : Constant  Value=apParams.mcLineJudge.segmentLimitRatio_f  OutDataTypeStr=single
  Constant5 : Constant  Value=apParams.trajGenParams.cruiseSpdNE_mps_f  OutDataTypeStr=single
  JudgeAlgorithm : MATLAB Function  TreatAsAtomicUnit=on
  JudgeAlgorithm1 : MATLAB Function  Commented=on  TreatAsAtomicUnit=on
  Selector : Selector  InputPortWidth=3  IndexOptions=Index vector (dialog)  Indices=[1 2]  OutputSizes=1
  Vector Concatenate : Concatenate
  Vector Concatenate1 : Concatenate
  Vector Concatenate2 : Concatenate
  mcLineJudge_b : Outport
  wires:
  JudgeAlgorithm/1(mcLineJudge_b) -> mcLineJudge_b/1
  Constant5/1 -> JudgeAlgorithm/5(maxRouteSpeed_mps_f)
  [maxAy_mps2_f] -> JudgeAlgorithm/6(maxLatAcc_mps2_f)
  Constant1/1 -> JudgeAlgorithm/7(minJudgeDist_m_f)
  Constant2/1 -> JudgeAlgorithm/8(maxJudgeDist_m_f)
  Constant3/1 -> JudgeAlgorithm/9(segmentLimitRatio_f)
  reset_b/1 -> JudgeAlgorithm/10(reset_b)
  Bus Selector/2 -> Vector Concatenate/2  "<posE_m_f>"
  Bus Selector/1 -> Vector Concatenate/1  "<posN_m_f>"
  preWp_struct/1 -> Bus Selector/1
  Vector Concatenate/1 -> [preWpNE_m_f]
  [preWpNE_m_f] -> JudgeAlgorithm/2(preWpNE_m_f)
  Bus Selector1/1 -> Vector Concatenate1/1  "<posN_m_f>"
  Bus Selector1/2 -> Vector Concatenate1/2  "<posE_m_f>"
  Vector Concatenate1/1 -> [curWpNE_m_f]
  curWp_struct/1 -> Bus Selector1/1
  [curWpNE_m_f] -> JudgeAlgorithm/3(curWpNE_m_f)
  [nextWpNE_m_f] -> JudgeAlgorithm/4(nextWpNE_m_f)
  Bus Selector2/1 -> Vector Concatenate2/1  "<posN_m_f>"
  Bus Selector2/2 -> Vector Concatenate2/2  "<posE_m_f>"
  Vector Concatenate2/1 -> [nextWpNE_m_f]
  nextWp_struct/1 -> Bus Selector2/1
  perfParams_struct/1 -> Bus Selector3/1
  Bus Selector3/1 -> Abs/1  "<maxAy_mps2_f>"
  Selector/1 -> JudgeAlgorithm/1(curPosNE_m_f)
  curPosNEU_m_f/1 -> Selector/1
  Abs/1 -> [maxAy_mps2_f]

== system GuidanceLaw/Subsystem/wpMssnHandle/GuiLaw/L1CirleGuidance/rollCmdLimit ==
  rollCmd_mps_f : Inport
  perfParams_struct : Inport  Port=2  OutDataTypeStr=Bus: perfParamBus
  curRoll_deg_f : Inport  Port=3
  reset_b : Inport  Port=4
  Add : Sum  Inputs=+-
  Add1 : Sum
  Bus Selector : BusSelector  OutputSignals=maxRollAngle_deg_f,minRollAngle_deg_f,maxRollAngleRate_dps_f,minRollAngleRate_dps_f
  Constant : Constant  Value=apParams.dt_s_f  OutDataTypeStr=single
  Constant1 : Constant  Value=apParams.dt_s_f  OutDataTypeStr=single
  Delay : Delay  DelayLength=1
  Product : Product
  Product1 : Product
  Saturation Dynamic : simulink/Discontinuities/Saturation Dynamic  OutMin=[]  OutMax=[]  OutDataTypeStr=Inherit: Same as second input  OutDataType=fixdt(1, 16)  OutScaling=2^-10  DoSatur=off
  Saturation Dynamic2 : simulink/Discontinuities/Saturation Dynamic  OutMin=[]  OutMax=[]  OutDataTypeStr=Inherit: Same as second input  OutDataType=fixdt(1, 16)  OutScaling=2^-10  DoSatur=off
  Switch : Switch  Criteria=u2 > Threshold  SaturateOnIntegerOverflow=off  InputSameDT=off
  rollCmdLimit_deg_f : Outport
  wires:
  [rollCmdPre_mps_f] -> Switch/3
  [reset_b] -> Switch/2
  [curRoll_deg_f] -> Switch/1
  Add/1 -> Saturation Dynamic/2
  Constant/1 -> Product/1
  Product/1 -> Saturation Dynamic/1
  Product1/1 -> Saturation Dynamic/3
  Constant1/1 -> Product1/2
  perfParams_struct/1 -> Bus Selector/1
  Bus Selector/1 -> [maxRollAngle_deg_f]  "<maxRollAngle_deg_f>"
  Bus Selector/2 -> [minRollAngle_deg_f]  "<minRollAngle_deg_f>"
  Bus Selector/3 -> [maxRollAngleRate_dps_f]  "<maxRollAngleRate_dps_f>"
  Bus Selector/4 -> [minRollAngleRate_dps_f]  "<minRollAngleRate_dps_f>"
  [maxRollAngleRate_dps_f] -> Product/2
  [minRollAngleRate_dps_f] -> Product1/1
  Saturation Dynamic/1 -> Add1/1
  rollCmd_mps_f/1 -> [rollCmd_mps_f]
  [rollCmd_mps_f] -> Add/1
  Add1/1 -> Saturation Dynamic2/2
  [maxRollAngle_deg_f] -> Saturation Dynamic2/1
  [minRollAngle_deg_f] -> Saturation Dynamic2/3
  Saturation Dynamic2/1 -> Delay/1, rollCmdLimit_deg_f/1
  Delay/1 -> [rollCmdPre_mps_f]
  curRoll_deg_f/1 -> [curRoll_deg_f]
  reset_b/1 -> [reset_b]
  Switch/1 -> Add/2, Add1/2

== system GuidanceLaw/Subsystem/wpMssnHandle/GuiLaw/L1LineGuidance/rollCmdLimit ==
  rollCmd_mps_f : Inport
  perfParams_struct : Inport  Port=2  OutDataTypeStr=Bus: perfParamBus
  curRoll_deg_f : Inport  Port=3
  reset_b : Inport  Port=4
  Add : Sum  Inputs=+-
  Add1 : Sum
  Bus Selector : BusSelector  OutputSignals=maxRollAngle_deg_f,minRollAngle_deg_f,maxRollAngleRate_dps_f,minRollAngleRate_dps_f
  Constant : Constant  Value=apParams.dt_s_f  OutDataTypeStr=single
  Constant1 : Constant  Value=apParams.dt_s_f  OutDataTypeStr=single
  Delay : Delay  DelayLength=1
  Product : Product
  Product1 : Product
  Saturation Dynamic : simulink/Discontinuities/Saturation Dynamic  OutMin=[]  OutMax=[]  OutDataTypeStr=Inherit: Same as second input  OutDataType=fixdt(1, 16)  OutScaling=2^-10  DoSatur=off
  Saturation Dynamic2 : simulink/Discontinuities/Saturation Dynamic  OutMin=[]  OutMax=[]  OutDataTypeStr=Inherit: Same as second input  OutDataType=fixdt(1, 16)  OutScaling=2^-10  DoSatur=off
  Switch : Switch  Criteria=u2 > Threshold  SaturateOnIntegerOverflow=off  InputSameDT=off
  rollCmdLimit_deg_f : Outport
  wires:
  [rollCmdPre_mps_f] -> Switch/3
  [reset_b] -> Switch/2
  [curRoll_deg_f] -> Switch/1
  Add/1 -> Saturation Dynamic/2
  Constant/1 -> Product/1
  Product/1 -> Saturation Dynamic/1
  Product1/1 -> Saturation Dynamic/3
  Constant1/1 -> Product1/2
  perfParams_struct/1 -> Bus Selector/1
  Bus Selector/1 -> [maxRollAngle_deg_f]  "<maxRollAngle_deg_f>"
  Bus Selector/2 -> [minRollAngle_deg_f]  "<minRollAngle_deg_f>"
  Bus Selector/3 -> [maxRollAngleRate_dps_f]  "<maxRollAngleRate_dps_f>"
  Bus Selector/4 -> [minRollAngleRate_dps_f]  "<minRollAngleRate_dps_f>"
  [maxRollAngleRate_dps_f] -> Product/2
  [minRollAngleRate_dps_f] -> Product1/1
  Saturation Dynamic/1 -> Add1/1
  rollCmd_mps_f/1 -> [rollCmd_mps_f]
  [rollCmd_mps_f] -> Add/1
  Add1/1 -> Saturation Dynamic2/2
  [maxRollAngle_deg_f] -> Saturation Dynamic2/1
  [minRollAngle_deg_f] -> Saturation Dynamic2/3
  Saturation Dynamic2/1 -> Delay/1, rollCmdLimit_deg_f/1
  Delay/1 -> [rollCmdPre_mps_f]
  curRoll_deg_f/1 -> [curRoll_deg_f]
  reset_b/1 -> [reset_b]
  Switch/1 -> Add1/2, Add/2

== system GuidanceLaw/Subsystem/wpMssnHandle/GuiLaw/invaildGuidance/NE2Body ==
  curYaw_deg_f : Inport  OutDataTypeStr=single
  curVn_mps_f : Inport  Port=2
  curVe_mps_f : Inport  Port=3
  Add : Sum
  Add1 : Sum
  Cos : Trigonometry  Operator=cos
  Degrees to Radians : simulink_extras/Transformations/Degrees to Radians
  Gain : Gain  Gain=-1
  Product{,1..3} (4 alike) : Product
  Sin : Trigonometry
  Sin1 : Trigonometry
  vxCmd_mps_f : Outport  OutDataTypeStr=single
  vyCmd_mps_f : Outport  Port=2  OutDataTypeStr=single
  wires:
  Product1/1 -> Add1/2
  Product2/1 -> Add/2
  [curYaw_deg_f] -> Degrees to Radians/1
  [curVe_mps_f] -> Product3/1
  Sin1/1 -> Product3/2
  Sin/1 -> Product2/1
  Product3/1 -> Add1/1
  Cos/1 -> Product1/2, Product/1
  Product/1 -> Add/1
  Degrees to Radians/1 -> Sin1/1, Sin/1, Cos/1
  Gain/1 -> Product2/2
  Add/1 -> vyCmd_mps_f/1
  [curVn_mps_f] -> Gain/1
  Add1/1 -> vxCmd_mps_f/1
  [curVn_mps_f] -> Product1/1
  [curVe_mps_f] -> Product/2
  curVn_mps_f/1 -> [curVn_mps_f]
  curVe_mps_f/1 -> [curVe_mps_f]
  curYaw_deg_f/1 -> [curYaw_deg_f]

== system GuidanceLaw/Subsystem/wpMssnHandle/GuiLaw/mcSpdGuidance/NE2Body ==
  curYaw_deg_f : Inport  OutDataTypeStr=single
  vnCmd_mps_f : Inport  Port=2
  veCmd_mps_f : Inport  Port=3
  Add : Sum
  Add1 : Sum
  Cos : Trigonometry  Operator=cos
  Degrees to Radians : simulink_extras/Transformations/Degrees to Radians
  Gain : Gain  Gain=-1
  Product{,1..3} (4 alike) : Product
  Sin : Trigonometry
  Sin1 : Trigonometry
  vxCmd_mps_f : Outport  OutDataTypeStr=single
  vyCmd_mps_f : Outport  Port=2  OutDataTypeStr=single
  wires:
  Product1/1 -> Add1/2
  Product2/1 -> Add/2
  [curYaw_deg_f] -> Degrees to Radians/1
  [veCmd_mps_f] -> Product3/1
  Sin1/1 -> Product3/2
  Sin/1 -> Product2/1
  Product3/1 -> Add1/1
  Cos/1 -> Product1/2, Product/1
  Product/1 -> Add/1
  Degrees to Radians/1 -> Sin1/1, Sin/1, Cos/1
  Gain/1 -> Product2/2
  Add/1 -> vyCmd_mps_f/1
  [vnCmd_mps_f] -> Gain/1
  Add1/1 -> vxCmd_mps_f/1
  [vnCmd_mps_f] -> Product1/1
  [veCmd_mps_f] -> Product/2
  vnCmd_mps_f/1 -> [vnCmd_mps_f]
  veCmd_mps_f/1 -> [veCmd_mps_f]
  curYaw_deg_f/1 -> [curYaw_deg_f]

== system GuidanceLaw/Subsystem/wpMssnHandle/GuiLaw/mcSpdGuidance/NE2Body1 ==
  curYaw_deg_f : Inport  OutDataTypeStr=single
  curVn_mps_f : Inport  Port=2
  curVe_mps_f : Inport  Port=3
  Add : Sum
  Add1 : Sum
  Cos : Trigonometry  Operator=cos
  Degrees to Radians : simulink_extras/Transformations/Degrees to Radians
  Gain : Gain  Gain=-1
  Product{,1..3} (4 alike) : Product
  Sin : Trigonometry
  Sin1 : Trigonometry
  curVx_mps_f : Outport  OutDataTypeStr=single
  curVy_mps_f : Outport  Port=2  OutDataTypeStr=single
  wires:
  Product1/1 -> Add1/2
  Product2/1 -> Add/2
  [curYaw_deg_f] -> Degrees to Radians/1
  [curVe_mps_f] -> Product3/1
  Sin1/1 -> Product3/2
  Sin/1 -> Product2/1
  Product3/1 -> Add1/1
  Cos/1 -> Product1/2, Product/1
  Product/1 -> Add/1
  Degrees to Radians/1 -> Sin1/1, Sin/1, Cos/1
  Gain/1 -> Product2/2
  Add/1 -> curVy_mps_f/1
  [curVn_mps_f] -> Gain/1
  Add1/1 -> curVx_mps_f/1
  [curVn_mps_f] -> Product1/1
  [curVe_mps_f] -> Product/2
  curVn_mps_f/1 -> [curVn_mps_f]
  curVe_mps_f/1 -> [curVe_mps_f]
  curYaw_deg_f/1 -> [curYaw_deg_f]

== system GuidanceLaw/Subsystem/wpMssnHandle/GuiLaw/mcSpdGuidance/mcHorizonPosGuidance ==
  trajPosNE_m_f : Inport
  trajVelNE_mps_f : Inport  Port=2
  posNE_m_f : Inport  Port=3
  perfParams_struct : Inport  Port=4  OutDataTypeStr=Bus: perfParamBus
  Bus Selector1 : BusSelector  OutputSignals=maxVx_mps_f
  Constant1 : Constant  Value=apParams.posGuiParams.kpE  OutDataTypeStr=single
  Constant11 : Constant  Value=apParams.posGuiParams.kpN  OutDataTypeStr=single
  Vector Concatenate : Concatenate
  horizonPosGuidance : MATLAB Function  TreatAsAtomicUnit=on
  velCmdNE_mps_f : Outport
  wires:
  horizonPosGuidance/1(velCmdNE_mps_f) -> velCmdNE_mps_f/1
  trajPosNE_m_f/1 -> [trajPosNE_m_f]
  trajVelNE_mps_f/1 -> [trajVelNE_mps_f]
  [trajPosNE_m_f] -> horizonPosGuidance/1(trajPosNE_m_f)
  [trajVelNE_mps_f] -> horizonPosGuidance/2(trajVelNE_mps_f)
  posNE_m_f/1 -> [posNE_m_f]
  [posNE_m_f] -> horizonPosGuidance/3(posNE_m_f)
  [maxVx_mps_f] -> horizonPosGuidance/5(maxVelNE_mps_f)
  Vector Concatenate/1 -> horizonPosGuidance/4(kpPosNE_per_s_f)
  Constant11/1 -> Vector Concatenate/1
  Constant1/1 -> Vector Concatenate/2
  perfParams_struct/1 -> [perfParams_struct]
  Bus Selector1/1 -> [maxVx_mps_f]  "<maxVx_mps_f>"
  [perfParams_struct] -> Bus Selector1/1

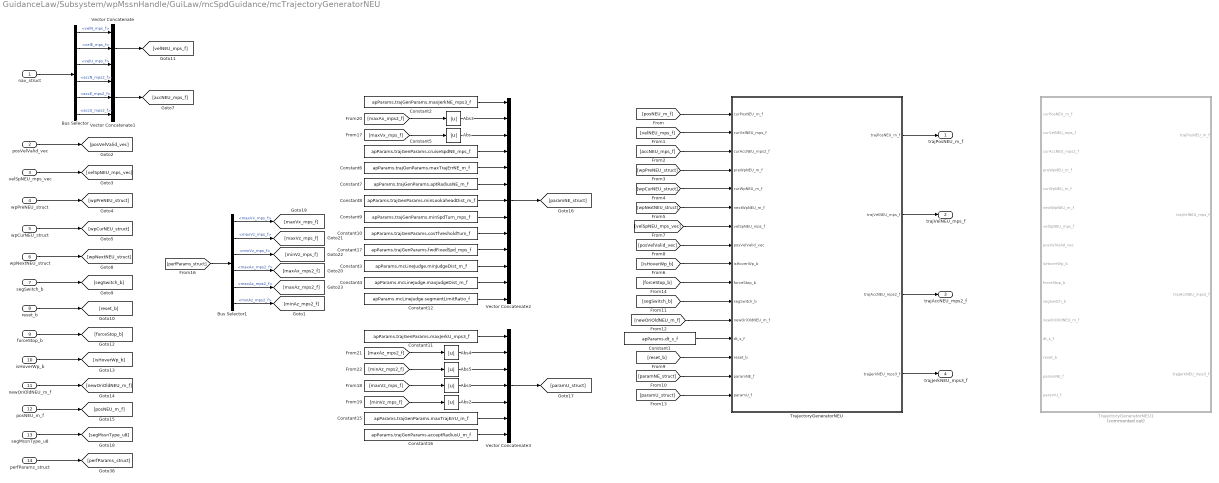
== system GuidanceLaw/Subsystem/wpMssnHandle/GuiLaw/mcSpdGuidance/mcTrajectoryGeneratorNEU ==
  nav_struct : Inport
  posVelValid_vec : Inport  Port=2
  velSpNEU_mps_vec : Inport  Port=3
  wpPreNEU_struct : Inport  Port=4
  wpCurNEU_struct : Inport  Port=5
  wpNextNEU_struct : Inport  Port=6
  segSwitch_b : Inport  Port=7
  reset_b : Inport  Port=8
  forceStop_b : Inport  Port=9
  isHoverWp_b : Inport  Port=10
  newOriOldNEU_m_f : Inport  Port=11
  posNEU_m_f : Inport  Port=12
  segMssnType_u8 : Inport  Port=13
  perfParams_struct : Inport  Port=14  OutDataTypeStr=Bus: perfParamBus
  Abs{,1..5} (6 alike) : Abs  SaturateOnIntegerOverflow=off
  Bus Selector : BusSelector  OutputSignals=velN_mps_f,velE_mps_f,velU_mps_f,accN_mps2_f,accE_mps2_f,accU_mps2_f
  Bus Selector1 : BusSelector  OutputSignals=maxVx_mps_f,maxVz_mps_f,minVz_mps_f,maxAx_mps2_f,maxAz_mps2_f,minAz_mps2_f
  Constant1 : Constant  Value=apParams.dt_s_f  OutDataTypeStr=single
  Constant10 : Constant  Value=apParams.trajGenParams.cosThresholdTurn_f  OutDataTypeStr=single
  Constant11 : Constant  Value=apParams.trajGenParams.maxJerkU_mps3_f  OutDataTypeStr=single
  Constant12 : Constant  Value=apParams.mcLineJudge.segmentLimitRatio_f  OutDataTypeStr=single
  Constant15 : Constant  Value=apParams.trajGenParams.maxTrajErrU_m_f  OutDataTypeStr=single
  Constant16 : Constant  Value=apParams.trajGenParams.acceptRadiusU_m_f  OutDataTypeStr=single
  Constant17 : Constant  Value=apParams.trajGenParams.fwdFixedSpd_mps_f  OutDataTypeStr=single
  Constant2 : Constant  Value=apParams.trajGenParams.maxJerkNE_mps3_f  OutDataTypeStr=single
  Constant3 : Constant  Value=apParams.mcLineJudge.minJudgeDist_m_f  OutDataTypeStr=single
  Constant4 : Constant  Value=apParams.mcLineJudge.maxJudgeDist_m_f  OutDataTypeStr=single
  Constant5 : Constant  Value=apParams.trajGenParams.cruiseSpdNE_mps_f  OutDataTypeStr=single
  Constant6 : Constant  Value=apParams.trajGenParams.maxTrajErrNE_m_f  OutDataTypeStr=single
  Constant7 : Constant  Value=apParams.trajGenParams.aptRadiusNE_m_f  OutDataTypeStr=single
  Constant8 : Constant  Value=apParams.trajGenParams.minLookaheadDist_m_f  OutDataTypeStr=single
  Constant9 : Constant  Value=apParams.trajGenParams.minSpdTurn_mps_f  OutDataTypeStr=single
  TrajectoryGeneratorNEU : MATLAB Function  TreatAsAtomicUnit=on
  TrajectoryGeneratorNEU1 : MATLAB Function  Commented=on  TreatAsAtomicUnit=on
  Vector Concatenate : Concatenate  NumInputs=3
  Vector Concatenate1 : Concatenate  NumInputs=3
  Vector Concatenate2 : Concatenate  NumInputs=13
  Vector Concatenate3 : Concatenate  NumInputs=7
  trajPosNEU_m_f : Outport
  trajVelNEU_mps_f : Outport  Port=2
  trajAccNEU_mps2_f : Outport  Port=3
  trajJerkNEU_mps3_f : Outport  Port=4
  wires:
  [posNEU_m_f] -> TrajectoryGeneratorNEU/1(curPosNEU_m_f)
  [velNEU_mps_f] -> TrajectoryGeneratorNEU/2(curVelNEU_mps_f)
  [accNEU_mps_f] -> TrajectoryGeneratorNEU/3(curAccNEU_mps2_f)
  [wpPreNEU_struct] -> TrajectoryGeneratorNEU/4(preWpNEU_m_f)
  [wpCurNEU_struct] -> TrajectoryGeneratorNEU/5(curWpNEU_m_f)
  [wpNextNEU_struct] -> TrajectoryGeneratorNEU/6(nextWpNEU_m_f)
  [isHoverWp_b] -> TrajectoryGeneratorNEU/9(isHoverWp_b)
  [forceStop_b] -> TrajectoryGeneratorNEU/10(forceStop_b)
  Constant1/1 -> TrajectoryGeneratorNEU/13(dt_s_f)
  [reset_b] -> TrajectoryGeneratorNEU/14(reset_b)
  [paramNE_struct] -> TrajectoryGeneratorNEU/15(paramNE_f)
  TrajectoryGeneratorNEU/4(trajJerkNEU_mps3_f) -> trajJerkNEU_mps3_f/1
  TrajectoryGeneratorNEU/3(trajAccNEU_mps2_f) -> trajAccNEU_mps2_f/1
  TrajectoryGeneratorNEU/2(trajVelNEU_mps_f) -> trajVelNEU_mps_f/1
  TrajectoryGeneratorNEU/1(trajPosNEU_m_f) -> trajPosNEU_m_f/1
  [segSwitch_b] -> TrajectoryGeneratorNEU/11(segSwitch_b)
  [newOriOldNEU_m_f] -> TrajectoryGeneratorNEU/12(newOriOldNEU_m_f)
  [paramU_struct] -> TrajectoryGeneratorNEU/16(paramU_f)
  nav_struct/1 -> Bus Selector/1
  Bus Selector/1 -> Vector Concatenate/1  "<velN_mps_f>"
  Bus Selector/2 -> Vector Concatenate/2  "<velE_mps_f>"
  Bus Selector/3 -> Vector Concatenate/3  "<velU_mps_f>"
  Vector Concatenate/1 -> [velNEU_mps_f]
  Bus Selector/4 -> Vector Concatenate1/1  "<accN_mps2_f>"
  Bus Selector/5 -> Vector Concatenate1/2  "<accE_mps2_f>"
  Bus Selector/6 -> Vector Concatenate1/3  "<accU_mps2_f>"
  Vector Concatenate1/1 -> [accNEU_mps_f]
  [velSpNEU_mps_vec] -> TrajectoryGeneratorNEU/7(velSpNEU_mps_f)
  [posVelValid_vec] -> TrajectoryGeneratorNEU/8(posVelValid_vec)
  posVelValid_vec/1 -> [posVelValid_vec]
  velSpNEU_mps_vec/1 -> [velSpNEU_mps_vec]
  wpPreNEU_struct/1 -> [wpPreNEU_struct]
  wpCurNEU_struct/1 -> [wpCurNEU_struct]
  wpNextNEU_struct/1 -> [wpNextNEU_struct]
  segSwitch_b/1 -> [segSwitch_b]
  reset_b/1 -> [reset_b]
  forceStop_b/1 -> [forceStop_b]
  isHoverWp_b/1 -> [isHoverWp_b]
  newOriOldNEU_m_f/1 -> [newOriOldNEU_m_f]
  posNEU_m_f/1 -> [posNEU_m_f]
  Constant2/1 -> Vector Concatenate2/1
  Abs3/1 -> Vector Concatenate2/2
  Abs/1 -> Vector Concatenate2/3
  Constant5/1 -> Vector Concatenate2/4
  Constant6/1 -> Vector Concatenate2/5
  Constant7/1 -> Vector Concatenate2/6
  Constant8/1 -> Vector Concatenate2/7
  Constant9/1 -> Vector Concatenate2/8
  Constant10/1 -> Vector Concatenate2/9
  Vector Concatenate2/1 -> [paramNE_struct]
  Vector Concatenate3/1 -> [paramU_struct]
  segMssnType_u8/1 -> [segMssnType_u8]
  Constant17/1 -> Vector Concatenate2/10
  perfParams_struct/1 -> [perfParams_struct]
  [perfParams_struct] -> Bus Selector1/1
  Bus Selector1/1 -> [maxVx_mps_f]  "<maxVx_mps_f>"
  Bus Selector1/4 -> [maxAx_mps2_f]  "<maxAx_mps2_f>"
  Bus Selector1/2 -> [maxVz_mps_f]  "<maxVz_mps_f>"
  Bus Selector1/3 -> [minVz_mps_f]  "<minVz_mps_f>"
  Bus Selector1/5 -> [maxAz_mps2_f]  "<maxAz_mps2_f>"
  [maxVx_mps_f] -> Abs/1
  [maxVz_mps_f] -> Abs1/1
  [minVz_mps_f] -> Abs2/1
  [maxAx_mps2_f] -> Abs3/1
  [maxAz_mps2_f] -> Abs4/1
  Bus Selector1/6 -> [minAz_mps2_f]  "<minAz_mps2_f>"
  Constant11/1 -> Vector Concatenate3/1
  Abs4/1 -> Vector Concatenate3/2
  Abs1/1 -> Vector Concatenate3/4
  Abs2/1 -> Vector Concatenate3/5
  Constant15/1 -> Vector Concatenate3/6
  Constant16/1 -> Vector Concatenate3/7
  [minAz_mps2_f] -> Abs5/1
  Abs5/1 -> Vector Concatenate3/3
  Constant3/1 -> Vector Concatenate2/11
  Constant4/1 -> Vector Concatenate2/12
  Constant12/1 -> Vector Concatenate2/13

== system GuidanceLaw/Subsystem/wpMssnHandle/GuiLaw/mcSpdGuidance/mcVertPosGuidance ==
  trajPosU_m_f : Inport
  curPosU_m_f : Inport  Port=2
  trajVu_mps_f : Inport  Port=3
  Add : Sum  Inputs=+-
  Add1 : Sum
  Constant : Constant  Value=apParams.posGuiParams.kpU  OutDataTypeStr=single
  Product : Product
  vuCmd_mps_f : Outport
  wires:
  [trajPosU_m_f] -> Add/1
  [curPosU_m_f] -> Add/2
  Add/1 -> Product/1
  Constant/1 -> Product/2
  Product/1 -> Add1/1
  [trajVu_mps_f] -> Add1/2
  Add1/1 -> vuCmd_mps_f/1
  curPosU_m_f/1 -> [curPosU_m_f]  "curPosU_m_f"
  trajPosU_m_f/1 -> [trajPosU_m_f]  "trajPosU_m_f"
  trajVu_mps_f/1 -> [trajVu_mps_f]  "trajVu_mps_f"
